simulink model "hrg_wa_v10_1_piezo"  (R2025a)
settings: Solver=FixedStepDiscrete  StartTime=0.0  StopTime=p.duration  FixedStep=p.Ts  RelTol=1e-3
model workspace (MAT data in the model file):
  Ad = [0.987688405123  -5.68131323296e-08  2.48971225508e-05  1.72406495467e-10  2.35500029057e-16  -7.48045553179e-18  2.39085041361e-17  1.59212234261e-22  0  0  0  0; 5.68131323296e-08  0.987688405123  -1.72406495467e-10  2.48971225508e-05  4.70881019476e-18  2.69344781657e-16  -1.59212235008e-22  2.39085041361e-17  0  0  0  0; -982.899001209  -0.00680633562581  0.987672737796  1.37356342331e-05  1.5611837146e-11  -5.09714578103e-13  9.88617178136e-13  1.31942511779e-17  0  0  0  0; 0.00680633562581  -982.899001209  -1.37356342331e-05  0.987672737796  3.12106539235e-13  1.83550880441e-11  -1.31942512097e-17  9.88617178136e-13  0  0  0  0; 0  0  0  0  0.28650479686  0  0  0  0  0  0  0; 0  0  0  0  0  0.352866081459  0  0  0  0  0  0; 943869.866875  6.2854468604  -988.617130951  -0.0131942506432  -1.52887962977e-08  4.97849569843e-10  -9.75634597461e-10  -1.26518662631e-14  0  0  0  0; -6.2854468604  943869.866875  0.0131942506432  -988.617130951  -3.05654153121e-10  -1.79275916498e-08  1.26518662949e-14  -9.75634597462e-10  0  0  0  0; 113668107.931  505.246320907  -239056.237822  -1.59199430864  -2.20191905684e-06  6.98200094534e-08  9.9975990594  -1.46549020767e-12  0.999750031247  0  0  0; -505.246320907  113668107.931  1.59199430864  -239056.237822  -4.4027695682e-08  -2.51395406668e-06  1.46549021355e-12  9.9975990594  0  0.999750031247  0  0; 62170953.3395  1554505.52703  -163920.493963  -4098.88409978  -1.27454644375e-06  4.00156404796e-09  9.50410725413  0.237602681353  0.956612237767  0.0239153059442  0.0432139182638  0; -882829.706009  61193845.2426  2356.91164918  -163353.073245  -7.00440355025e-09  -1.4233603888e-06  -0.139969993764  9.70458623439  -0.0141100303999  0.97829544106  0  0.0591645112941]
  Bd = [1.07541978092e-16  -2.80909408987e-18; 2.15044631223e-18  1.01140599362e-16; 1.17750014529e-11  -3.11685647158e-13; 2.35440509738e-13  1.12226992357e-11; 0.71349520314  0; 0  0.647133918541; -1.10105605369e-08  2.90941885987e-10; -2.20157780066e-10  -1.04757152027e-08; -9.65252715165e-07  2.517993119e-08; -1.93016562843e-08  -9.06591565342e-07; -4.58609339763e-07  1.18833226824e-09; -2.49830556256e-09  -4.18846719335e-07]
  c.detect = [-9972404109.88+545531236.399i  -249309643.885+13636860.8122i; 149494718.172-9008065.32861i  -10364964237.4+624623483.105i]
  c.sample_period_s = 2.5e-05
  c.drive = [1.0677844451e-06-2.20398878536e-07i  -3.17521469995e-08+7.37540079324e-09i; 2.13555769115e-08-4.4075121339e-09i  1.14308554761e-06-2.65485352229e-07i]
  c.nominal_detect = -9999678898.08+46914376.8426i
  p.schema = 'v10.1'
  p.synthetic = 1
  p.f0 = 1000
  p.gamma_intrinsic = 0.314159265359
  p.Cs = 1e-09
  p.G0 = 1e-10
  p.kappa = 1e-06
  p.b = 1.1e-06
  p.Cds = 0
  p.Rs = 1000
  p.B = 0.276990961962
  p.Omega = 0.5
  p.Ts = 2.5e-05
  p.Tc = 0.001
  p.duration = 0.8
  p.charge_target = 1e-11
  p.initial_fraction = 0.3
  p.theta0 = 0.4
  p.Cf = 1e-10
  p.Rf = 1000000000
  p.driver_tau = [2e-05; 2.4e-05]
  p.afe_bw = [20000; 18000]
  p.detect_matrix = [1  0.025; -0.015  1.04]
  p.drive_matrix = [1  -0.03; 0.02  1.08]
  p.split_hz = 0
  p.stiffness_axis = 0.37
  p.damping_half_difference = 0
  p.damping_axis = -0.23
  p.adc_span = 2
  p.adc_bits = 20
  p.dac_span = 2
  p.dac_bits = 18
  p.vmax = 1
  p.agc_bw = 5
  p.quad_bw = 4
  p.pll_gain = 30
  p.max_detune = 30
  p.virtual_rate = 0
  p.virtual_start_min_s = 0.25
  p.virtual_settle_fraction = 0.01
  p.predict_heading = 1
  p.max_heading_rate = 100
  p.virtual_validated_limit = 0.2
  p.min_amplitude_fraction = 0.02
  p.min_linearity = 0.1
  p.max_calibration_condition = 100
  p.max_frame_age = 0.002
  p.calibrate_detection = 1
  p.calibrate_drive = 1
  p.noise_rms_V = 0
  p.noise_seed = 20261030
  plant_p.schema = 'v10.1'
  plant_p.synthetic = 1
  plant_p.f0 = 1000
  plant_p.gamma_intrinsic = 0.314159265359
  plant_p.Cs = 1e-09
  plant_p.G0 = 1e-10
  plant_p.kappa = 1e-06
  plant_p.b = 1.1e-06
  plant_p.Cds = 0
  plant_p.Rs = 1000
  plant_p.B = 0.276990961962
  plant_p.Omega = 0.5
  plant_p.Ts = 2.5e-05
  plant_p.Tc = 0.001
  plant_p.duration = 0.8
  plant_p.charge_target = 1e-11
  plant_p.initial_fraction = 0.3
  plant_p.theta0 = 0.4
  plant_p.Cf = 1e-10
  plant_p.Rf = 1000000000
  plant_p.driver_tau = [2e-05; 2.4e-05]
  plant_p.afe_bw = [20000; 18000]
  plant_p.detect_matrix = [1  0.025; -0.015  1.04]
  plant_p.drive_matrix = [1  -0.03; 0.02  1.08]
  plant_p.split_hz = 0
  plant_p.stiffness_axis = 0.37
  plant_p.damping_half_difference = 0
  plant_p.damping_axis = -0.23
  plant_p.adc_span = 2
  plant_p.adc_bits = 20
  plant_p.dac_span = 2
  plant_p.dac_bits = 18
  plant_p.vmax = 1
  plant_p.agc_bw = 5
  plant_p.quad_bw = 4
  plant_p.pll_gain = 30
  plant_p.max_detune = 30
  plant_p.virtual_rate = 0
  plant_p.virtual_start_min_s = 0.25
  plant_p.virtual_settle_fraction = 0.01
  plant_p.predict_heading = 1
  plant_p.max_heading_rate = 100
  plant_p.virtual_validated_limit = 0.2
  plant_p.min_amplitude_fraction = 0.02
  plant_p.min_linearity = 0.1
  plant_p.max_calibration_condition = 100
  plant_p.max_frame_age = 0.002
  plant_p.calibrate_detection = 1
  plant_p.calibrate_drive = 1
  plant_p.noise_rms_V = 0
  plant_p.noise_seed = 20261030
  x0 = [2.76318298201e-12; 1.16825502693e-12; 0; 0; 0; 0; 0; 0; 0; 0; 0; 0]
Description:
  | V10.1 synthetic motional-charge carrier loop. Intrinsic mechanical damping + explicit electrical load. Window-center timestamps, angle validity, independent calibration profile, integer-domain DAC clipping.
settings Model: Creator=11725  LastModifiedBy=11725

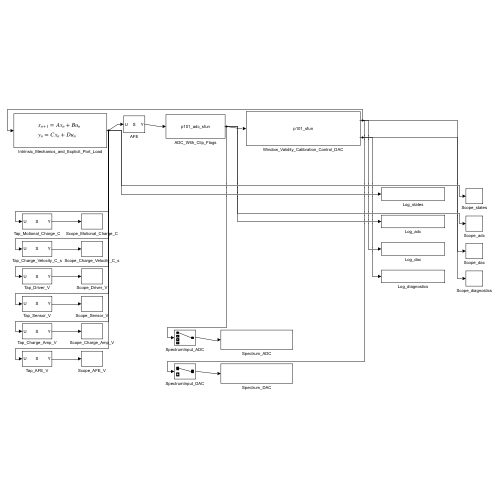
[thumbnail: Simulink's stored preview of the top-level diagram]
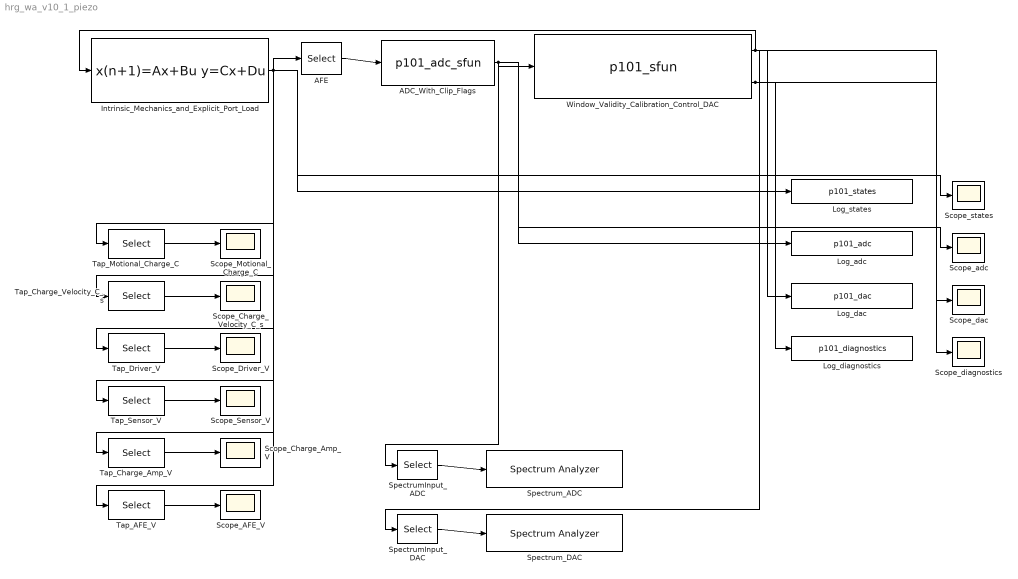
== system hrg_wa_v10_1_piezo ==
  ADC_With_Clip_Flags : M-S-Function  FunctionName=p101_adc_sfun  Parameters=p
  AFE : Selector  InputPortWidth=12  IndexOptions=Index vector (dialog)  Indices=[11 12]  OutputSizes=1
  Intrinsic_Mechanics_and_Explicit_Port_Load : DiscreteStateSpace  A=Ad  B=Bd  C=eye(12)  D=zeros(12,2)  InitialCondition=x0  SampleTime=p.Ts
  Log_adc : ToWorkspace  VariableName=p101_adc  SaveFormat=Timeseries  SampleTime=-1
  Log_dac : ToWorkspace  VariableName=p101_dac  SaveFormat=Timeseries  SampleTime=-1
  Log_diagnostics : ToWorkspace  VariableName=p101_diagnostics  SaveFormat=Timeseries  SampleTime=-1
  Log_states : ToWorkspace  VariableName=p101_states  SaveFormat=Timeseries  SampleTime=-1
  Scope_AFE_V : Scope
  Scope_Charge_Amp_V : Scope
  Scope_Charge_Velocity_C_s : Scope
  Scope_Driver_V : Scope
  Scope_Motional_Charge_C : Scope
  Scope_Sensor_V : Scope
  Scope_adc : Scope
  Scope_dac : Scope
  Scope_diagnostics : Scope
  Scope_states : Scope
  SpectrumInput_ADC : Selector  InputPortWidth=4  IndexOptions=Index vector (dialog)  Indices=1  OutputSizes=1
  SpectrumInput_DAC : Selector  InputPortWidth=2  IndexOptions=Index vector (dialog)  Indices=1  OutputSizes=1
  Spectrum_ADC : SpectrumAnalyzer  SampleRateSource=Property  SampleRate=40000  WindowInvariantSamplesPerUpdate=on  SpectrumUnits=dBV
      settings: OpenAtSimulationStart=off
  Spectrum_DAC : SpectrumAnalyzer  SampleRateSource=Property  SampleRate=40000  WindowInvariantSamplesPerUpdate=on  SpectrumUnits=dBV
      settings: OpenAtSimulationStart=off
  Tap_AFE_V : Selector  InputPortWidth=12  IndexOptions=Index vector (dialog)  Indices=[11 12]  OutputSizes=1
  Tap_Charge_Amp_V : Selector  InputPortWidth=12  IndexOptions=Index vector (dialog)  Indices=[9 10]  OutputSizes=1
  Tap_Charge_Velocity_C_s : Selector  InputPortWidth=12  IndexOptions=Index vector (dialog)  Indices=[3 4]  OutputSizes=1
  Tap_Driver_V : Selector  InputPortWidth=12  IndexOptions=Index vector (dialog)  Indices=[5 6]  OutputSizes=1
  Tap_Motional_Charge_C : Selector  InputPortWidth=12  IndexOptions=Index vector (dialog)  Indices=[1 2]  OutputSizes=1
  Tap_Sensor_V : Selector  InputPortWidth=12  IndexOptions=Index vector (dialog)  Indices=[7 8]  OutputSizes=1
  Window_Validity_Calibration_Control_DAC : M-S-Function  FunctionName=p101_sfun  Parameters=p,c
  wires:
  Intrinsic_Mechanics_and_Explicit_Port_Load/1 -> AFE/1, Log_states/1, Scope_states/1, Tap_Motional_Charge_C/1, Tap_Charge_Velocity_C_s/1, Tap_Driver_V/1, Tap_Sensor_V/1, Tap_Charge_Amp_V/1, Tap_AFE_V/1
  AFE/1 -> ADC_With_Clip_Flags/1
  ADC_With_Clip_Flags/1 -> Window_Validity_Calibration_Control_DAC/1, Log_adc/1, Scope_adc/1, SpectrumInput_ADC/1
  Window_Validity_Calibration_Control_DAC/1 -> Intrinsic_Mechanics_and_Explicit_Port_Load/1, Log_dac/1, Scope_dac/1, SpectrumInput_DAC/1
  Window_Validity_Calibration_Control_DAC/2 -> Log_diagnostics/1, Scope_diagnostics/1
  Tap_Motional_Charge_C/1 -> Scope_Motional_Charge_C/1
  Tap_Charge_Velocity_C_s/1 -> Scope_Charge_Velocity_C_s/1
  Tap_Driver_V/1 -> Scope_Driver_V/1
  Tap_Sensor_V/1 -> Scope_Sensor_V/1
  Tap_Charge_Amp_V/1 -> Scope_Charge_Amp_V/1
  Tap_AFE_V/1 -> Scope_AFE_V/1
  SpectrumInput_ADC/1 -> Spectrum_ADC/1
  SpectrumInput_DAC/1 -> Spectrum_DAC/1
